simulink model "gnc_StatusMetrics"  (R2026b)
settings: Solver=VariableStepAuto
values from neighbouring files (symbols this model uses):
  Ts = prm.Ts    [gnc_missionFSM.m]    (also in gnc_mpcPlantUpdate.m)
  xte = (abx*(py - qy) - aby*(px - qx))/nab    [gnc_pathAnalyzer.m]
undefined symbols (not defined in the file or in its folder): area_done_m2, AutoSub, dist_home, eta_s, fault_word, gnc_state, GncState, heading_err, hold_reason, hold_timer, mission_done, mission_id, mission_type, n_seg, nav_ok, P, PathSrc, pause_reason, pose_est, progress, replan_count, seg_idx, soc_rth, sub_mode, tracker_active, v_ref, xte_rms
libraries: simulink x3, dspstat3 x1, dspmathops x1, sl_discontinuities x1
settings Model: Creator=aomar  LastModifiedBy=aomar

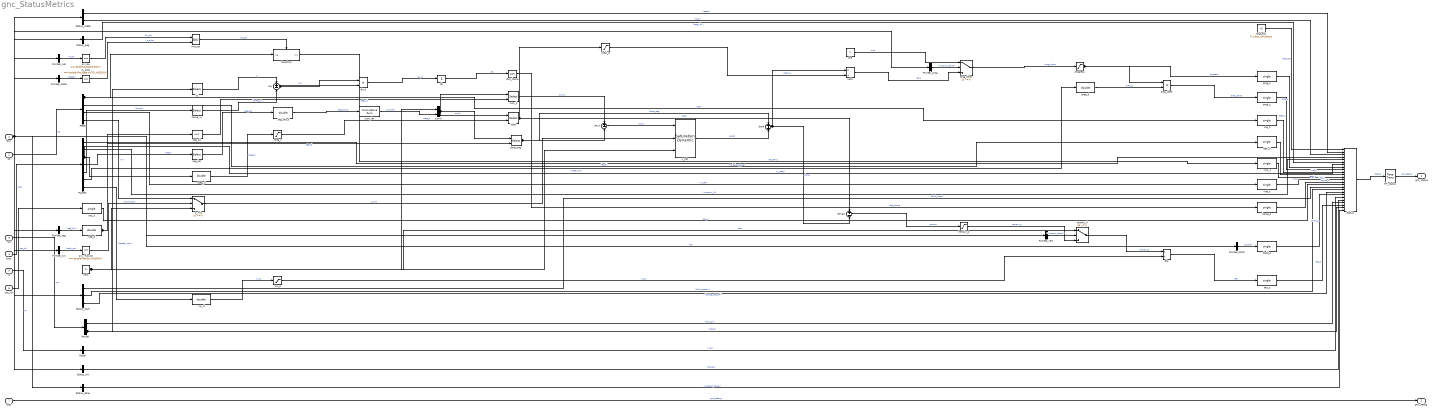
== system gnc_StatusMetrics ==
  fsm : Inport  OutDataTypeStr=Bus: Bus_FsmOut  SampleTime=Ts.gnc
  pe : Inport  Port=2  OutDataTypeStr=Bus: Bus_PathError  SampleTime=Ts.gnc
  nav : Inport  Port=3  OutDataTypeStr=Bus: Bus_NavCond  SampleTime=Ts.gnc
  plan : Inport  Port=4  OutDataTypeStr=Bus: Bus_MissionPlan
  rp : Inport  Port=5  OutDataTypeStr=Bus: Bus_ReplanResult  SampleTime=Ts.gnc
  soc_rth : Inport  Port=6  OutDataTypeStr=double  PortDimensions=1  SampleTime=Ts.gnc
  dbg : Inport  Port=7  OutDataTypeStr=Bus: Bus_GncDebug  SampleTime=Ts.gnc
  FsmSel_prog : BusSelector  OutputSignals=mission_done
  FsmSel_rem : BusSelector  OutputSignals=mission_done
  FsmSel_seg : BusSelector  OutputSignals=seg_idx
  FsmSel_src : BusSelector  OutputSignals=path_src
  FsmSel_state : BusSelector  OutputSignals=state
  FsmSel_sub : BusSelector  OutputSignals=sub
  FsmSel_thold : BusSelector  OutputSignals=t_hold
  NavSel : BusSelector  OutputSignals=nav_ok,pose
  PeSel : BusSelector  OutputSignals=xte,epsi,v_ref,s
  PlanSel : BusSelector  OutputSignals=mission_type,mission_id,n_seg,seg,home,area_m2,speed_work
  RT_status : RateTransition  OutPortSampleTime=Ts.gnc_status
  RowRms : Subsystem  TreatAsAtomicUnit=on
  RpSel : BusSelector  OutputSignals=ver
  Status : BusAssignment  AssignedSignals=gnc_state,sub_mode,mission_type,mission_id,seg_idx,n_seg,progress,area_done_m2,xte,heading_err,xte_rms,v_ref,dist_home,soc_rth,fault_word,hold_reason,pause_reason,hold_timer,replan_count,tracker_active,nav_ok,eta_s,pose_est,mission_done
  StatusIC : Constant  Value=P.ic.Bus_GncStatus  OutDataTypeStr=Bus: Bus_GncStatus  SampleTime=Ts.gnc
  Status_done : BusSelector  OutputSignals=mission_done
  Status_fault : BusSelector  OutputSignals=fault_word,hold_reason,pause_reason
  Status_seg : BusSelector  OutputSignals=seg_idx
  Status_state : BusSelector  OutputSignals=state,sub
  Status_trk : BusSelector  OutputSignals=trk_sel
  area_d : DataTypeConversion  OutDataTypeStr=double  RndMeth=Nearest
  area_done : Product  Inputs=**
  area_s : DataTypeConversion  OutDataTypeStr=single  RndMeth=Nearest
  cum0 : Concatenate
  cum_k : Selector  IndexOptions=Index vector (port)  OutputSizes=1
  cum_len : dspmathops/Cumulative Sum  dim=Columns  InputProcessing=Columns as channels (frame based)  reset_popup=None  roundingMode=Floor  overflowMode=off  outputDataTypeStr=Inherit: Same as accumulator  outputMin=[]  outputMax=[]  outputLastDataTypeStr=Inherit: Same as accumulator
  d2 : Sum  Inputs=+
  dist_home : Sqrt
  done : Sum
  done_seg : Selector  IndexOptions=Index vector (port)  OutputSizes=1
  dxy : Sum  Inputs=+-
  dxy2 : Product  Inputs=**
  epsi_s : DataTypeConversion  OutDataTypeStr=single  RndMeth=Nearest
  eta : Product  Inputs=*/
  eta_s : DataTypeConversion  OutDataTypeStr=single  RndMeth=Nearest
  home_s : DataTypeConversion  OutDataTypeStr=single  RndMeth=Nearest
  home_xy : Selector  IndexOptions=Index vector (dialog)  Indices=[1 2]  OutputSizes=1
  is_auto : simulink/Logic and Bit Operations/Compare To Constant  relop===  const=double(GncState.AUTO_MISSION)  OutDataTypeStr=boolean
  len_k : Sum  Inputs=+-
  nseg_c : Saturate  UpperLimit=P.gnc.path.S_max  LowerLimit=1
  nseg_d : DataTypeConversion  OutDataTypeStr=double  RndMeth=Nearest
  on_row : simulink/Logic and Bit Operations/Compare To Constant  relop===  const=double(AutoSub.ROW)  OutDataTypeStr=boolean
  one : Constant  OutDataTypeStr=double  SampleTime=Ts.gnc
  prog_done : Switch  Criteria=u2 ~= 0  SaturateOnIntegerOverflow=off  InputSameDT=off
  prog_s : DataTypeConversion  OutDataTypeStr=single  RndMeth=Nearest
  progress : Saturate  UpperLimit=1  LowerLimit=0
  ratio : Product  Inputs=*/
  remain : Sum  Inputs=+-
  remain_d : Switch  Criteria=u2 ~= 0  SaturateOnIntegerOverflow=off  InputSameDT=off
  remain_p : Saturate  UpperLimit=inf  LowerLimit=0
  rms_en : Logic  AllPortsSameDT=off  OutDataTypeStr=boolean
  rms_s : DataTypeConversion  OutDataTypeStr=single  RndMeth=Nearest
  s_mis : Switch  Criteria=u2 ~= 0  SaturateOnIntegerOverflow=off  InputSameDT=off
  s_pos : sl_discontinuities/Saturation Dynamic  OutMin=[]  OutMax=[]  OutDataTypeStr=Inherit: Same as second input  OutDataType=fixdt(1, 16)  OutScaling=2^-10  DoSatur=off
      settings: LibrarySourceBlock=|
      | simulink/Discontinuities/Saturation
      | Dynamic
  seg_d : DataTypeConversion  OutDataTypeStr=double  RndMeth=Nearest
  seg_len : Selector  NumberOfDimensions=2  InputPortWidth=3  IndexOptions=Select all,Index vector (dialog)  Indices=,3  OutputSizes=1
  seg_len_d : DataTypeConversion  OutDataTypeStr=double  RndMeth=Nearest
  seg_p1 : Bias  Bias=1  SaturateOnIntegerOverflow=off
  soc_s : DataTypeConversion  OutDataTypeStr=single  RndMeth=Nearest
  src_mission : simulink/Logic and Bit Operations/Compare To Constant  relop===  const=double(PathSrc.MISSION)  OutDataTypeStr=boolean
  thold_s : DataTypeConversion  OutDataTypeStr=single  RndMeth=Nearest
  total : Selector  IndexOptions=Index vector (port)  OutputSizes=1
  total_p : Saturate  UpperLimit=inf  LowerLimit=1e-6
  vref_s : DataTypeConversion  OutDataTypeStr=single  RndMeth=Nearest
  vw_d : DataTypeConversion  OutDataTypeStr=double  RndMeth=Nearest
  vw_p : Saturate  UpperLimit=inf  LowerLimit=P.gnc.met.v_eta_min
  xte_s : DataTypeConversion  OutDataTypeStr=single  RndMeth=Nearest
  xy : Selector  IndexOptions=Index vector (dialog)  Indices=[1 2]  OutputSizes=1
  zero : Constant  Value=0  OutDataTypeStr=double  SampleTime=Ts.gnc
  gnc_status : Outport  OutDataTypeStr=Bus: Bus_GncStatus
  gnc_debug : Outport  Port=2  OutDataTypeStr=Bus: Bus_GncDebug
  wires:
  fsm/1 -> Status_done/1, Status_trk/1, Status_fault/1, Status_state/1, FsmSel_src/1, FsmSel_thold/1, FsmSel_rem/1, Status_seg/1, FsmSel_seg/1, FsmSel_sub/1, FsmSel_prog/1, FsmSel_state/1  "fsm"
  pe/1 -> PeSel/1  "pe"
  nav/1 -> NavSel/1  "nav"
  plan/1 -> PlanSel/1  "plan"
  rp/1 -> RpSel/1  "rp"
  soc_rth/1 -> soc_s/1  "soc_rth"
  dbg/1 -> gnc_debug/1  "gnc_debug"
  FsmSel_sub/1 -> on_row/1  "<sub>"
  FsmSel_state/1 -> is_auto/1  "<state>"
  FsmSel_seg/1 -> seg_d/1  "<seg_idx>"
  FsmSel_src/1 -> src_mission/1  "<path_src>"
  Status_state/1 -> Status/2  "<state>"
  Status_state/2 -> Status/3  "<sub>"
  Status_seg/1 -> Status/6  "<seg_idx>"
  PeSel/1 -> RowRms/1(xte), xte_s/1  "<xte>"
  PeSel/2 -> epsi_s/1  "<epsi>"
  PeSel/3 -> vref_s/1  "<v_ref>"
  PeSel/4 -> s_mis/1  "<s>"
  PlanSel/1 -> Status/4  "<mission_type>"
  PlanSel/2 -> Status/5  "<mission_id>"
  PlanSel/5 -> home_xy/1  "<home>"
  PlanSel/6 -> area_d/1  "<area_m2>"
  PlanSel/7 -> vw_d/1  "<speed_work>"
  Status_fault/1 -> Status/16  "<fault_word>"
  Status_fault/2 -> Status/17  "<hold_reason>"
  Status_fault/3 -> Status/18  "<pause_reason>"
  RpSel/1 -> Status/20  "<ver>"
  Status_trk/1 -> Status/21  "<trk_sel>"
  Status_done/1 -> Status/25  "<mission_done>"
  NavSel/1 -> Status/22  "<nav_ok>"
  NavSel/2 -> xy/1, Status/24  "<pose>"
  on_row/1 -> rms_en/1  "on_row"
  is_auto/1 -> rms_en/2  "is_auto"
  src_mission/1 -> s_mis/2  "src_mission"
  zero/1 -> cum0/1, s_pos/3, s_mis/3, remain_d/1  "zero"
  soc_s/1 -> Status/15  "soc_s"
  seg_d/1 -> seg_p1/1, done_seg/2  "seg_d"
  rms_en/1 -> RowRms/Enable  "rms_en"
  xy/1 -> dxy/1  "xy"
  home_xy/1 -> dxy/2  "home_xy"
  seg_p1/1 -> cum_k/2  "seg_p1"
  seg_len/1 -> seg_len_d/1  "seg_len"
  s_mis/1 -> s_pos/2  "s_mis"
  nseg_d/1 -> nseg_c/1  "nseg_d"
  vw_d/1 -> vw_p/1  "vw_d"
  dxy/1 -> dxy2/1, dxy2/2  "dxy"
  nseg_c/1 -> total/2  "nseg_c"
  vw_p/1 -> eta/2  "vw_p"
  seg_len_d/1 -> cum_len/1  "seg_len_d"
  RowRms/1(rms) -> rms_s/1  "RowRms"
  dxy2/1 -> d2/1  "dxy2"
  cum_len/1 -> cum0/2  "cum_len"
  cum0/1 -> done_seg/1, cum_k/1, total/1  "cum0"
  d2/1 -> dist_home/1  "d2"
  dist_home/1 -> home_s/1  "dist_home"
  cum_k/1 -> len_k/1  "cum_k"
  total/1 -> remain/1, total_p/1  "total"
  done_seg/1 -> done/1, len_k/2  "done_seg"
  len_k/1 -> s_pos/1  "len_k"
  total_p/1 -> ratio/2  "total_p"
  s_pos/1 -> done/2  "s_pos"
  done/1 -> remain/2, ratio/1  "done"
  remain/1 -> remain_p/1  "remain"
  one/1 -> prog_done/1  "one"
  ratio/1 -> prog_done/3  "ratio"
  FsmSel_prog/1 -> prog_done/2  "<mission_done>"
  remain_p/1 -> remain_d/3  "remain_p"
  prog_done/1 -> progress/1  "prog_done"
  FsmSel_rem/1 -> remain_d/2  "<mission_done>"
  progress/1 -> area_done/1, prog_s/1  "progress"
  remain_d/1 -> eta/1  "remain_d"
  area_d/1 -> area_done/2  "area_d"
  area_done/1 -> area_s/1  "area_done"
  eta/1 -> eta_s/1  "eta"
  FsmSel_thold/1 -> thold_s/1  "<t_hold>"
  StatusIC/1 -> Status/1  "StatusIC"
  prog_s/1 -> Status/8  "prog_s"
  area_s/1 -> Status/9  "area_s"
  xte_s/1 -> Status/10  "xte_s"
  epsi_s/1 -> Status/11  "epsi_s"
  rms_s/1 -> Status/12  "rms_s"
  vref_s/1 -> Status/13  "vref_s"
  home_s/1 -> Status/14  "home_s"
  thold_s/1 -> Status/19  "thold_s"
  eta_s/1 -> Status/23  "eta_s"
  Status/1 -> RT_status/1  "Status"
  RT_status/1 -> gnc_status/1  "gnc_status"
  PlanSel/3 -> nseg_d/1, Status/7  "<n_seg>"
  PlanSel/4 -> seg_len/1  "<seg>"

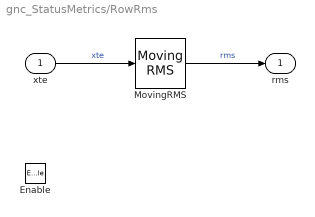
== system gnc_StatusMetrics/RowRms ==
  xte : Inport
  Enable : EnablePort
  MovingRMS : dspstat3/Moving RMS  Method=Sliding window  ForgettingFactorPort=off  SpecifyWindowLength=on  EnableTunableWindowLength=off  WindowLengthFromInputPort=off  TunableWindowLength=4  MaxWindowLength=20  AutoAdjustInvalidWindowLength=on  WindowLength=P.gnc.met.rms_window  OverlapLength=P.gnc.met.rms_window - 1  AllowArbitraryInputLength=off  ForgettingFactor=0.9  SimulateUsing=Code generation
  rms : Outport  InitialOutput=0
  wires:
  xte/1 -> MovingRMS/1  "xte"
  MovingRMS/1 -> rms/1  "rms"
